simulink model "course_lab4_reduced"  (R2024b)
settings: Solver=ode45  StartTime=0.0  StopTime=4  MaxStep=0.002666666666666667  RelTol=1e-7  AbsTol=1e-9
model workspace (MAT data in the model file):
  A = 1
  K = 1
  T1 = 0.1
  T2 = 0.1
  den = [0.1 1 10]
  frequency = 1
  num = [0 0 10]
  web_input = timeseries
  web_input.Name = 'unnamed'
  web_input.DataInfo = tsdata.datametadata
  web_input.DataInfo.Interpolation = tsdata.interpolation
  web_input.DataInfo.Interpolation.Fhandle : function handle (value not decoded)
  web_input.DataInfo.Interpolation.Name = 'linear'
  web_input.TimeInfo = tsdata.timemetadata
  web_input.TimeInfo.Length = 1501
  web_input.TimeInfo.DuplicateTimes = 0
  web_input.TimeInfo.Time_ = [0 0.00266666666667 0.00533333333333 0.008 0.0106666666667 0.0133333333333 0.016 0.0186666666667 0.0213333333333 0.024 0.0266666666667 0.0293333333333 ... (1501 elements, 1501x1)]
  web_input.TimeInfo.Initialized = 1
  web_input.QualityInfo = tsdata.qualmetadata
  web_input.Data_ = [1 1 1 1 1 1 1 1 1 1 1 1 ... (1501 elements, 1501x1)]
settings Model: Creator=33657  LastModifiedBy=33657

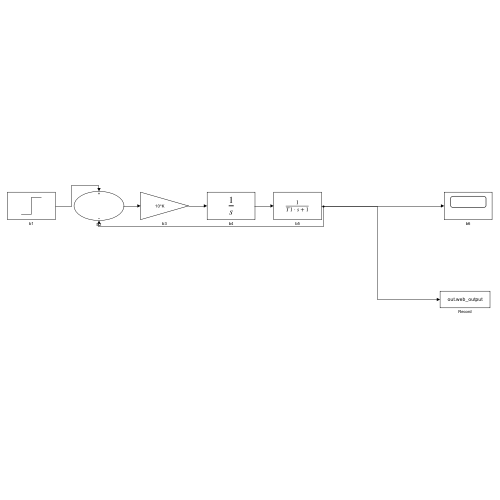
[thumbnail: Simulink's stored preview of the top-level diagram]
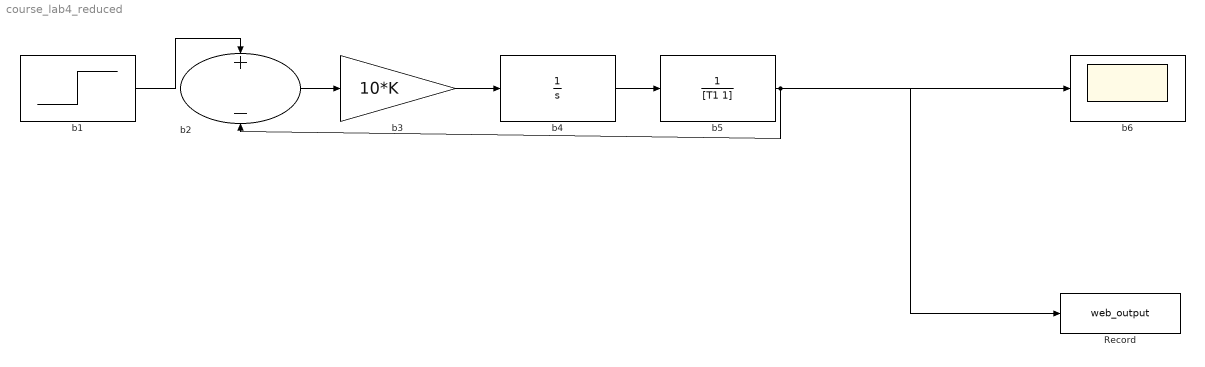
== system course_lab4_reduced ==
  Record : ToWorkspace  VariableName=web_output  SaveFormat=Timeseries  SampleTime=-1
  b1 : Step  Time=0  After=A  SampleTime=0
  b2 : Sum  Inputs=+-
  b3 : Gain  Gain=10*K
  b4 : Integrator
  b5 : TransferFcn  Denominator=[T1 1]
  b6 : Scope
  wires:
  b1/1 -> b2/1
  b2/1 -> b3/1
  b3/1 -> b4/1
  b4/1 -> b5/1
  b5/1 -> b2/2, b6/1, Record/1
